simulink model "StarshipSystemModel"  (R2025b)
settings: Solver=VariableStepAuto  StartTime=0.0  StopTime=10.0  RelTol=1e-3
model workspace (MAT data in the model file):
  ActiveGNCMode : Simulink.Bus (value not decoded)
  AerodynamicControlCommand : Simulink.Bus (value not decoded)
  AerodynamicLoad : Simulink.Bus (value not decoded)
  AggregatedStream : Simulink.Bus (value not decoded)
  AllocatedEffectorDemand : Simulink.Bus (value not decoded)
  AttitudeControlDemand : Simulink.Bus (value not decoded)
  AttitudeGuidanceCommand : Simulink.Bus (value not decoded)
  AttitudeRateState : Simulink.Bus (value not decoded)
  AutogenousPressurantGas : Simulink.ConnectionBus (value not decoded)
  CandidateFaultIndication : Simulink.Bus (value not decoded)
  CombustionGasFeed : Simulink.ConnectionBus (value not decoded)
  CommandPathHealth : Simulink.Bus (value not decoded)
  ControlMode : Simulink.ValueType (value not decoded)
  DownlinkSignal : Simulink.Bus (value not decoded)
  ElectricalPower : Simulink.ConnectionBus (value not decoded)
  EngineTelemetry : Simulink.Bus (value not decoded)
  ExecutionContext : Simulink.Bus (value not decoded)
  FaultDiagnosisResult : Simulink.Bus (value not decoded)
  GNCDataContext : Simulink.Bus (value not decoded)
  GNCHealthState : Simulink.Bus (value not decoded)
  GNCStateEstimate : Simulink.Bus (value not decoded)
  GimbalAngle : Simulink.ValueType (value not decoded)
  GimbalMotion : Simulink.ConnectionBus (value not decoded)
  GroundCheckoutLink : Simulink.Bus (value not decoded)
  GroundPressurantSupply : Simulink.ConnectionBus (value not decoded)
  GuidanceConstraints : Simulink.Bus (value not decoded)
  GuidanceMode : Simulink.ValueType (value not decoded)
  LinkHealth : Simulink.Bus (value not decoded)
  LiquidPropellantFeed : Simulink.ConnectionBus (value not decoded)
  MechanicalMotion : Simulink.ConnectionBus (value not decoded)
  MechanismPosition : Simulink.Bus (value not decoded)
  ModeTransitionContext : Simulink.Bus (value not decoded)
  NavigationAidingData : Simulink.Bus (value not decoded)
  NavigationEstimate : Simulink.Bus (value not decoded)
  NavigationHealthStatus : Simulink.Bus (value not decoded)
  NavigationMeasurementSet : Simulink.Bus (value not decoded)
  PercentThrottle : Simulink.ValueType (value not decoded)
  PneumaticActuationGas : Simulink.ConnectionBus (value not decoded)
  PowerConversionStatus : Simulink.Bus (value not decoded)
  PowerDistributionStatus : Simulink.Bus (value not decoded)
  PowerHealthStatus : Simulink.Bus (value not decoded)
  PowerManagementCommand : Simulink.Bus (value not decoded)
  PowerStorageStatus : Simulink.Bus (value not decoded)
  ProtectedThermalState : Simulink.Bus (value not decoded)
  ProtectionIsolationStatus : Simulink.Bus (value not decoded)
  PurgeGasSupply : Simulink.ConnectionBus (value not decoded)
  RCSPulseCommand : Simulink.Bus (value not decoded)
  RCSTelemetry : Simulink.Bus (value not decoded)
  RFFeed : Simulink.ConnectionBus (value not decoded)
  RecoveryMechanismCommand : Simulink.Bus (value not decoded)
  RollThrottleBias : Simulink.ValueType (value not decoded)
  SafetyOverride : Simulink.ValueType (value not decoded)
  SafetyStateStatus : Simulink.Bus (value not decoded)
  ShapedControlDemand : Simulink.Bus (value not decoded)
  SpinStartIgniterGas : Simulink.ConnectionBus (value not decoded)
  StageMechanicalBoundary : Simulink.ConnectionBus (value not decoded)
  StructuralLoad : Simulink.ConnectionBus (value not decoded)
  StructureHealthStatus : Simulink.Bus (value not decoded)
  SubsystemHealthEvidence : Simulink.Bus (value not decoded)
  SubsystemStatusTelemetry : Simulink.Bus (value not decoded)
  TankTelemetry : Simulink.Bus (value not decoded)
  ThermalMonitoringCommand : Simulink.Bus (value not decoded)
  ThermalNetwork : Simulink.ConnectionBus (value not decoded)
  ThrustLoad : Simulink.ConnectionBus (value not decoded)
  TrajectoryGuidanceCommand : Simulink.Bus (value not decoded)
  TrajectoryReference : Simulink.Bus (value not decoded)
  TranslationalControlDemand : Simulink.Bus (value not decoded)
  TranslationalState : Simulink.Bus (value not decoded)
  UplinkSignal : Simulink.Bus (value not decoded)
  ValidatedControlDemand : Simulink.Bus (value not decoded)
  ValveCommand : Simulink.ValueType (value not decoded)
  VehicleStructureState : Simulink.Bus (value not decoded)
  VerifiedCommand : Simulink.Bus (value not decoded)
  VideoStream : Simulink.Bus (value not decoded)
undefined symbols (not defined in the file): ACR, ACT, ASM, ATM, BCR, BDQ, BDR, BDX, BEC, BFC, BHV, BIP, BLM, BNZ, BPI, BPR, BPV, BRX, BSM, BTA, BTP, BVC, BVE, BVV, CAA, CAM, CAS, CAT, CLM, COM, CRS, CTL, CTR, DAQ, ESC, EXT, FCR, FDB, FDE, FEX, FHI, FHM, FIC, FIS, FMG, FSC, GAP, GCM, GMD, GNC, GND, GPH, GTR, HDN, HIA, HSI, IF, INT, LOC, NAI ... (+45)
(part 8 of 8)

== system StarshipSystemModel/Starship/Propulsion/Booster main engines/Engine controller ==
  Bus Element In1 : Inport  PortName=IF-GNC-BEC-01
  Bus Element In2 : Inport  Port=2  PortName=IF-SAF-BEC-01
  IF-PWR-BEC-01 : PMIOPort  Side=Left  ConnectionType=Bus: ElectricalPower
  Bus Element Out1 : Outport  PortName=IF-BEC-SAF-01
  Bus Element Out2 : Outport  Port=2  PortName=IF-BEC-BTA-01
  Bus Element Out3 : Outport  Port=3  PortName=IF-BEC-BVC-01

== system StarshipSystemModel/Starship/Propulsion/Booster main engines/Ignition system ==
  IF-BIG-BPB-01 : PMIOPort  Side=Right
  IF-BSG-BIG-01 : PMIOPort  Port=2  Side=Left  ConnectionType=Bus: SpinStartIgniterGas

== system StarshipSystemModel/Starship/Propulsion/Booster main engines/Mounting interface ==
  IF-GMB-BMT-01 : PMIOPort  Side=Left  ConnectionType=Bus: GimbalMotion
  IF-BMT-TLI-01 : PMIOPort  Port=2  Side=Right  ConnectionType=Bus: StructuralLoad

== system StarshipSystemModel/Starship/Propulsion/Booster main engines/Nozzle ==
  IF-BCC-BNZ-01 : PMIOPort  Side=Left  ConnectionType=Bus: CombustionGasFeed
  Bus Element Out1 : Outport  PortName=IF-BNZ-BTP-01

== system StarshipSystemModel/Starship/Propulsion/Booster main engines/Preburners ==
  IF-BTP-BPB-01 : PMIOPort  Side=Left  ConnectionType=Bus: CombustionGasFeed
  IF-BPB-BCC-01 : PMIOPort  Port=2  Side=Right  ConnectionType=Bus: CombustionGasFeed
  IF-BIG-BPB-01 : PMIOPort  Port=3  Side=Left

== system StarshipSystemModel/Starship/Propulsion/Booster main engines/Turbopumps ==
  IF-BDM-BTP-01 : PMIOPort  Side=Left  ConnectionType=Bus: LiquidPropellantFeed
  IF-BVC-BTP-01 : PMIOPort  Port=2  Side=Left  ConnectionType=Bus: LiquidPropellantFeed
  IF-BTP-BPR-01 : PMIOPort  Port=3  Side=Right  ConnectionType=Bus: AutogenousPressurantGas
  IF-BTP-BPB-01 : PMIOPort  Port=4  Side=Right  ConnectionType=Bus: CombustionGasFeed

== system StarshipSystemModel/Starship/Propulsion/Booster main engines/Valves & control ==
  Bus Element In1 : Inport  PortName=IF-BEC-BVC-01
  IF-BVC-BTP-01 : PMIOPort  Side=Right  ConnectionType=Bus: LiquidPropellantFeed
  IF-BNG-BVC-01 : PMIOPort  Port=2  Side=Left  ConnectionType=Bus: PneumaticActuationGas

== system StarshipSystemModel/Starship/Propulsion/Gimbal // TVC actuation/Gimbal bearing ==
  IF-YAC-GMB-01 : PMIOPort  Side=Left  ConnectionType=Bus: GimbalMotion
  IF-PAC-GMB-01 : PMIOPort  Port=2  Side=Left  ConnectionType=Bus: GimbalMotion
  IF-GMB-BMT-01 : PMIOPort  Port=3  Side=Right  ConnectionType=Bus: GimbalMotion
  IF-GMB-SMT-01 : PMIOPort  Port=4  Side=Right  ConnectionType=Bus: GimbalMotion

== system StarshipSystemModel/Starship/Propulsion/Gimbal // TVC actuation/Pitch actuator ==
  Bus Element In1 : Inport  PortName=IF-TVC-PAC-01
  IF-PAC-GMB-01 : PMIOPort  Side=Right  ConnectionType=Bus: GimbalMotion

== system StarshipSystemModel/Starship/Propulsion/Gimbal // TVC actuation/TVC controller ==
  Bus Element In1 : Inport  PortName=IF-GNC-TVC-01
  IF-PWR-TVC-01 : PMIOPort  Side=Left  ConnectionType=Bus: ElectricalPower
  Bus Element Out1 : Outport  PortName=IF-TVC-GNC-01
  Bus Element Out3 : Outport  Port=2  PortName=IF-TVC-YAC-01
  Bus Element Out2 : Outport  Port=3  PortName=IF-TVC-PAC-01

== system StarshipSystemModel/Starship/Propulsion/Gimbal // TVC actuation/Yaw actuator ==
  Bus Element In1 : Inport  PortName=IF-TVC-YAC-01
  IF-YAC-GMB-01 : PMIOPort  Side=Right  ConnectionType=Bus: GimbalMotion

== system StarshipSystemModel/Starship/Propulsion/RCS thrusters/Igniter ==
  IF-RIG-RTC-01 : PMIOPort  Side=Right

== system StarshipSystemModel/Starship/Propulsion/RCS thrusters/RCS controller ==
  Bus Element In1 : Inport  PortName=IF-GNC-RCT-01
  IF-PWR-RCT-01 : PMIOPort  Side=Left  ConnectionType=Bus: ElectricalPower
  Bus Element Out1 : Outport  PortName=IF-RCT-SAF-01
  Bus Element Out2 : Outport  Port=2  PortName=IF-RCT-RVM-01

== system StarshipSystemModel/Starship/Propulsion/RCS thrusters/Thruster chamber, nozzle ==
  IF-RVM-RTC-01 : PMIOPort  Side=Left  ConnectionType=Bus: CombustionGasFeed
  IF-RIG-RTC-01 : PMIOPort  Port=2  Side=Left

== system StarshipSystemModel/Starship/Propulsion/RCS thrusters/Valve & feed manifold ==
  Bus Element In1 : Inport  PortName=IF-RCT-RVM-01
  IF-SPR-RVM-01 : PMIOPort  Side=Left  ConnectionType=Bus: CombustionGasFeed
  IF-RVM-RTC-01 : PMIOPort  Port=2  Side=Right  ConnectionType=Bus: CombustionGasFeed

== system StarshipSystemModel/Starship/Propulsion/Ship main engines/Combustion Chamber  ==
  IF-SPB-SCC-01 : PMIOPort  Side=Left  ConnectionType=Bus: CombustionGasFeed
  IF-SCC-SNZ-01 : PMIOPort  Port=2  Side=Right  ConnectionType=Bus: CombustionGasFeed

== system StarshipSystemModel/Starship/Propulsion/Ship main engines/Engine controller ==
  Bus Element In1 : Inport  PortName=IF-GNC-SEC-01
  Bus Element In2 : Inport  Port=2  PortName=IF-SAF-SEC-01
  IF-PWR-SEC-01 : PMIOPort  Side=Left  ConnectionType=Bus: ElectricalPower
  Bus Element Out1 : Outport  PortName=IF-SEC-SAF-01
  Bus Element Out2 : Outport  Port=2  PortName=IF-SEC-STA-01
  Bus Element Out3 : Outport  Port=3  PortName=IF-SEC-SVC-01

== system StarshipSystemModel/Starship/Propulsion/Ship main engines/Ignition system ==
  IF-SIG-SPB-01 : PMIOPort  Side=Right
  IF-SSG-SIG-01 : PMIOPort  Port=2  Side=Left  ConnectionType=Bus: SpinStartIgniterGas

== system StarshipSystemModel/Starship/Propulsion/Ship main engines/Mounting interface ==
  IF-GMB-SMT-01 : PMIOPort  Side=Left  ConnectionType=Bus: GimbalMotion
  IF-SMT-TLI-01 : PMIOPort  Port=2  Side=Right  ConnectionType=Bus: StructuralLoad

== system StarshipSystemModel/Starship/Propulsion/Ship main engines/Nozzle ==
  IF-SCC-SNZ-01 : PMIOPort  Side=Left  ConnectionType=Bus: CombustionGasFeed
  Bus Element Out1 : Outport  PortName=IF-SNZ-STP-01

== system StarshipSystemModel/Starship/Propulsion/Ship main engines/Preburners ==
  IF-STP-SPB-01 : PMIOPort  Side=Left  ConnectionType=Bus: CombustionGasFeed
  IF-SIG-SPB-01 : PMIOPort  Port=2  Side=Left
  IF-SPB-SCC-01 : PMIOPort  Port=3  Side=Right  ConnectionType=Bus: CombustionGasFeed

== system StarshipSystemModel/Starship/Propulsion/Ship main engines/Turbopumps ==
  IF-SDM-STP-01 : PMIOPort  Side=Left  ConnectionType=Bus: LiquidPropellantFeed
  IF-SVC-STP-01 : PMIOPort  Port=2  Side=Left  ConnectionType=Bus: LiquidPropellantFeed
  IF-STP-SPR-01 : PMIOPort  Port=3  Side=Right  ConnectionType=Bus: AutogenousPressurantGas
  IF-STP-SPB-01 : PMIOPort  Port=4  Side=Right  ConnectionType=Bus: CombustionGasFeed

== system StarshipSystemModel/Starship/Propulsion/Ship main engines/Valves & control ==
  Bus Element In1 : Inport  PortName=IF-SEC-SVC-01
  IF-SVC-STP-01 : PMIOPort  Side=Right  ConnectionType=Bus: LiquidPropellantFeed
  IF-SNG-SVC-01 : PMIOPort  Port=2  Side=Left  ConnectionType=Bus: PneumaticActuationGas

== system StarshipSystemModel/Starship/Safety & Fault Management /Fault Diagnosis & Isolation/Fault Correlation & Reasoning ==
  Bus Element In1 : Inport  PortName=IF-FDE-FCR-01
  Bus Element Out1 : Outport  PortName=IF-FCR-FIS-01

== system StarshipSystemModel/Starship/Safety & Fault Management /Fault Diagnosis & Isolation/Fault Identification & Classification ==
  Bus Element In1 : Inport  PortName=IF-FIS-FIC-01
  Bus Element Out1 : Outport  PortName=IF-FIC-SEA-01

== system StarshipSystemModel/Starship/Safety & Fault Management /Fault Diagnosis & Isolation/Fault Isolation ==
  Bus Element In1 : Inport  PortName=IF-FCR-FIS-01
  Bus Element Out1 : Outport  PortName=IF-FIS-FIC-01

== system StarshipSystemModel/Starship/Safety & Fault Management /Fault Management & Response Logic/Protective Action Coordination ==
  Bus Element In1 : Inport  PortName=IF-RSL-PAC-01
  Bus Element Out1 : Outport  PortName=IF-SAF-BEC-01
  Bus Element Out2 : Outport  Port=2  PortName=IF-SAF-SEC-01
  Bus Element Out3 : Outport  Port=3  PortName=IF-PAC-RCO-01

== system StarshipSystemModel/Starship/Safety & Fault Management /Fault Management & Response Logic/Response Selection Logic ==
  Bus Element In1 : Inport  PortName=IF-SEA-RSL-01
  Bus Element Out1 : Outport  PortName=IF-RSL-PAC-01

== system StarshipSystemModel/Starship/Safety & Fault Management /Fault Management & Response Logic/Severity & Consequence Assessment ==
  Bus Element In1 : Inport  PortName=IF-FIC-SEA-01
  Bus Element Out1 : Outport  PortName=IF-SEA-RSL-01

== system StarshipSystemModel/Starship/Safety & Fault Management /Health Monitoring & Fault Detection/Fault Detection Engine ==
  Bus Element In1 : Inport  PortName=IF-VIE-FDE-01
  Bus Element Out1 : Outport  PortName=IF-FDE-FCR-01

== system StarshipSystemModel/Starship/Safety & Fault Management /Health Monitoring & Fault Detection/Health Information Aggregation ==
  Bus Element In11 : Inport  PortName=IF-RSM-SAF-01
  Bus Element In10 : Inport  Port=2  PortName=IF-INT-SAF-01
  Bus Element In9 : Inport  Port=3  PortName=IF-POS-SAF-01
  Bus Element In8 : Inport  Port=4  PortName=IF-TMS-SAF-01
  Bus Element In7 : Inport  Port=5  PortName=IF-FHM-SAF-01
  Bus Element In1 : Inport  Port=6  PortName=IF-BEC-SAF-01
  Bus Element In2 : Inport  Port=7  PortName=IF-SEC-SAF-01
  Bus Element In3 : Inport  Port=8  PortName=IF-RCT-SAF-01
  Bus Element In4 : Inport  Port=9  PortName=IF-BPR-SAF-01
  Bus Element In5 : Inport  Port=10  PortName=IF-SPR-SAF-01
  Bus Element In6 : Inport  Port=11  PortName=IF-PMM-SAF-01
  Bus Element In12 : Inport  Port=12  PortName=IF-BLM-SAF-01
  Bus Element In13 : Inport  Port=13  PortName=IF-SLM-SAF-01
  Bus Element In14 : Inport  Port=14  PortName=IF-ESC-HIA-01
  Bus Element Out1 : Outport  PortName=IF-HIA-VIE-01

== system StarshipSystemModel/Starship/Safety & Fault Management /Health Monitoring & Fault Detection/Validity & Integrity Evaluation ==
  Bus Element In1 : Inport  PortName=IF-HIA-VIE-01
  Bus Element Out1 : Outport  PortName=IF-VIE-FDE-01

== system StarshipSystemModel/Starship/Safety & Fault Management /Recovery & Reconfiguration Management/Reconfiguration Coordinator ==
  Bus Element In1 : Inport  PortName=IF-PAC-RCO-01
  Bus Element Out1 : Outport  PortName=IF-RCO-RSE-01

== system StarshipSystemModel/Starship/Safety & Fault Management /Recovery & Reconfiguration Management/Recovery Sequence Executor ==
  Bus Element In1 : Inport  PortName=IF-RCO-RSE-01
  Bus Element Out1 : Outport  PortName=IF-SAF-RSM-01
  Bus Element Out2 : Outport  Port=2  PortName=IF-RSE-RVF-01

== system StarshipSystemModel/Starship/Safety & Fault Management /Recovery & Reconfiguration Management/Recovery Verification ==
  Bus Element In1 : Inport  PortName=IF-RSE-RVF-01
  Bus Element Out1 : Outport  PortName=IF-RVF-SSM-01

== system StarshipSystemModel/Starship/Safety & Fault Management /Safety State & Flight-Safety Management/Escalation & Containment Status ==
  Bus Element In1 : Inport  PortName=IF-FSC-ESC-01
  Bus Element Out2 : Outport  PortName=IF-SAF-STA-01
  Bus Element Out1 : Outport  Port=2  PortName=IF-SAF-BTA-01
  Bus Element Out3 : Outport  Port=3  PortName=IF-ESC-HIA-01

== system StarshipSystemModel/Starship/Safety & Fault Management /Safety State & Flight-Safety Management/Flight-Safety Coordination ==
  Bus Element In1 : Inport  PortName=IF-BCR-SAF-01
  Bus Element In2 : Inport  Port=2  PortName=IF-SCR-SAF-01
  Bus Element In3 : Inport  Port=3  PortName=IF-SSM-FSC-01
  Bus Element Out1 : Outport  PortName=IF-FSC-ESC-01

== system StarshipSystemModel/Starship/Safety & Fault Management /Safety State & Flight-Safety Management/Safety State Manager ==
  Bus Element In1 : Inport  PortName=IF-RVF-SSM-01
  Bus Element Out1 : Outport  PortName=IF-SAF-FHM-01
  Bus Element Out2 : Outport  Port=2  PortName=IF-SSM-FSC-01

== system StarshipSystemModel/Starship/Structure and Mechanisms/Aerodynamic Control Mechanisms/Actuator ==
  Bus Element In1 : Inport  PortName=IF-GNC-ACT-01
  Bus Element In2 : Inport  Port=2  PortName=IF-POS-ACT-01
  IF-ACT-HNG-01 : PMIOPort  Side=Right  ConnectionType=Bus: MechanicalMotion
  IF-PWR-STR-01 : PMIOPort  Port=2  Side=Left  ConnectionType=Bus: ElectricalPower

== system StarshipSystemModel/Starship/Structure and Mechanisms/Aerodynamic Control Mechanisms/Hinge // linkage ==
  IF-SUR-HNG-01 : PMIOPort  Side=Left  ConnectionType=Bus: MechanicalMotion
  IF-ACT-HNG-01 : PMIOPort  Port=2  Side=Left  ConnectionType=Bus: MechanicalMotion
  IF-HNG-SUR-01 : PMIOPort  Port=3  Side=Right
  IF-HNG-INT-01 : PMIOPort  Port=4  Side=Right

== system StarshipSystemModel/Starship/Structure and Mechanisms/Aerodynamic Control Mechanisms/Position // health ==
  Bus Element Out1 : Outport  PortName=IF-POS-GNC-01
  Bus Element Out2 : Outport  Port=2  PortName=IF-POS-ACT-01
  Bus Element Out3 : Outport  Port=3  PortName=IF-POS-SAF-01

== system StarshipSystemModel/Starship/Structure and Mechanisms/Aerodynamic Control Mechanisms/Surface // fin // flap ==
  Bus Element In1 : Inport  PortName=IF-ATM-SUR-01
  IF-HNG-SUR-01 : PMIOPort  Side=Left
  IF-SUR-HNG-01 : PMIOPort  Port=2  Side=Right  ConnectionType=Bus: MechanicalMotion

== system StarshipSystemModel/Starship/Structure and Mechanisms/Primary Load-Bearing Airframe/ Load-transfer structure ==
  IF-PRS-LDT-01 : PMIOPort  Side=Left
  IF-LDT-INT-01 : PMIOPort  Port=2  Side=Right
  IF-TLI-LDT-01 : PMIOPort  Port=3  Side=Left

== system StarshipSystemModel/Starship/Structure and Mechanisms/Primary Load-Bearing Airframe/Local interface structure ==
  IF-LDT-INT-01 : PMIOPort  Side=Left
  IF-INT-PRS-01 : PMIOPort  Port=2  Side=Right
  IF-SLS-LDT-01 : PMIOPort  Port=3  Side=Left
  IF-HNG-INT-01 : PMIOPort  Port=4  Side=Left
  Bus Element Out3 : Outport  PortName=IF-INT-SAF-01
  Bus Element Out1 : Outport  Port=2  PortName=IF-INT-STA-01
  Bus Element Out2 : Outport  Port=3  PortName=IF-INT-BTA-01

== system StarshipSystemModel/Starship/Structure and Mechanisms/Primary Load-Bearing Airframe/Primary pressure//shell ==
  IF-BOT-PRS-01 : PMIOPort  Side=Right  ConnectionType=Bus: StructuralLoad
  IF-SOT-PRS-01 : PMIOPort  Port=2  Side=Right  ConnectionType=Bus: StructuralLoad
  IF-RLI-PRS-01 : PMIOPort  Port=3  Side=Left
  IF-TBI-PRS-01 : PMIOPort  Port=4  Side=Left  ConnectionType=Bus: ThermalNetwork
  IF-BTP-PRS-01 : PMIOPort  Port=5  Side=Left  ConnectionType=Bus: ThermalNetwork
  IF-STP-PRS-01 : PMIOPort  Port=6  Side=Left  ConnectionType=Bus: ThermalNetwork
  IF-PRS-LDT-01 : PMIOPort  Port=7  Side=Right
  IF-INT-PRS-01 : PMIOPort  Port=8  Side=Left

== system StarshipSystemModel/Starship/Structure and Mechanisms/Recovery & Landing Mechanisms/Landing//catch load path ==
  IF-RLI-GND-01 : PMIOPort  Side=Right  ConnectionType=Bus: StructuralLoad
  IF-RME-RLI-01 : PMIOPort  Port=2  Side=Left  ConnectionType=Bus: MechanicalMotion
  IF-RLI-PRS-01 : PMIOPort  Port=3  Side=Right

== system StarshipSystemModel/Starship/Structure and Mechanisms/Recovery & Landing Mechanisms/Recovery mechanism ==
  IF-RME-RLI-01 : PMIOPort  Side=Right  ConnectionType=Bus: MechanicalMotion
  Bus Element Out1 : Outport  PortName=IF-RME-RSM-01

== system StarshipSystemModel/Starship/Structure and Mechanisms/Recovery & Landing Mechanisms/Recovery state//health ==
  Bus Element In1 : Inport  PortName=IF-RME-RSM-01
  Bus Element In2 : Inport  Port=2  PortName=IF-SAF-RSM-01
  Bus Element Out1 : Outport  PortName=IF-RSM-SAF-01

== system StarshipSystemModel/Starship/Structure and Mechanisms/Stage & Thrust Interfaces/Hot-stage interface ==
  IF-HSI-SLS-01 : PMIOPort  Side=Right  ConnectionType=Bus: StageMechanicalBoundary

== system StarshipSystemModel/Starship/Structure and Mechanisms/Stage & Thrust Interfaces/Separation response ==
  IF-HSI-SLS-01 : PMIOPort  Side=Left  ConnectionType=Bus: StageMechanicalBoundary
  IF-SLS-LDT-01 : PMIOPort  Port=2  Side=Right

== system StarshipSystemModel/Starship/Structure and Mechanisms/Stage & Thrust Interfaces/Thrust-load introduction ==
  IF-BMT-TLI-01 : PMIOPort  Side=Right
  IF-SMT-TLI-01 : PMIOPort  Port=2  Side=Right
  IF-TLI-LDT-01 : PMIOPort  Port=3  Side=Right

== system StarshipSystemModel/Starship/Thermal Protection/Ship Primary TPS/Base heat-shield region ==

== system StarshipSystemModel/Starship/Thermal Protection/Ship Primary TPS/Control-surface thermal protection ==
  Bus Element Out1 : Outport  PortName=IF-STP-CTL-TBI-CTL-01

== system StarshipSystemModel/Starship/Thermal Protection/Ship Primary TPS/Localized high-heating protection ==
  Bus Element Out1 : Outport  PortName=IF-STP-LOC-TBI-STP-01

== system StarshipSystemModel/Starship/Thermal Protection/Ship Primary TPS/Primary TPS acreage // tile field ==
  Bus Element In1 : Inport  PortName=IF-ATM-STP-01
  Bus Element In2 : Inport  Port=2  PortName=IF-SNZ-STP-01
  IF-STP-PRS-01 : PMIOPort  Side=Right  ConnectionType=Bus: ThermalNetwork
  Bus Element Out1 : Outport  PortName=IF-STP-ACR-TBI-GAP-01

== system StarshipSystemModel/Starship/Thermal Protection/Super Heavy Thermal Protection/Base heat-shield region ==

== system StarshipSystemModel/Starship/Thermal Protection/Super Heavy Thermal Protection/Forward heat-shield // interstage ==
  Bus Element Out1 : Outport  PortName=IF-BTP-FHI-TBI-INT-01

== system StarshipSystemModel/Starship/Thermal Protection/Super Heavy Thermal Protection/Localized thermal protection ==
  IF-BTP-PRS-01 : PMIOPort  Side=Right  ConnectionType=Bus: ThermalNetwork
  Bus Element Out1 : Outport  PortName=IF-BTP-LOC-TBI-STP-01

== system StarshipSystemModel/Starship/Thermal Protection/Super Heavy Thermal Protection/Primary TPS acreage ==
  Bus Element In1 : Inport  PortName=IF-BNZ-BTP-01
  Bus Element In2 : Inport  Port=2  PortName=IF-ATM-BTP-01
  Bus Element Out1 : Outport  PortName=IF-BTP-ACR-TBI-GAP-01

== system StarshipSystemModel/Starship/Thermal Protection/Thermal Barriers & Discontinuity Protection/Control-surface boundary // closeout protection ==
  Bus Element In1 : Inport  PortName=IF-STP-CTL-TBI-CTL-01
  Bus Element Out1 : Outport  PortName=IF-TBI-CTL-TMS-SNS-01

== system StarshipSystemModel/Starship/Thermal Protection/Thermal Barriers & Discontinuity Protection/Penetration and interface barriers ==
  Bus Element In1 : Inport  PortName=IF-BTP-FHI-TBI-INT-01
  Bus Element Out1 : Outport  PortName=IF-TBI-INT-TMS-SNS-01

== system StarshipSystemModel/Starship/Thermal Protection/Thermal Barriers & Discontinuity Protection/Step // protrusion thermal management ==
  Bus Element In2 : Inport  PortName=IF-BTP-LOC-TBI-STP-01
  Bus Element In1 : Inport  Port=2  PortName=IF-STP-LOC-TBI-STP-01
  IF-TBI-PRS-01 : PMIOPort  Side=Right  ConnectionType=Bus: ThermalNetwork

== system StarshipSystemModel/Starship/Thermal Protection/Thermal Barriers & Discontinuity Protection/Tile-gap // seam thermal protection ==
  Bus Element In2 : Inport  PortName=IF-BTP-ACR-TBI-GAP-01
  Bus Element In1 : Inport  Port=2  PortName=IF-STP-ACR-TBI-GAP-01
  Bus Element Out1 : Outport  PortName=IF-TBI-GAP-TMS-SNS-01

== system StarshipSystemModel/Starship/Thermal Protection/Thermal Monitoring & Assessment/External thermal-observation data interface ==
  Bus Element Out1 : Outport  PortName=IF-TMS-EXT-ASM-01

== system StarshipSystemModel/Starship/Thermal Protection/Thermal Monitoring & Assessment/TPS thermal sensors ==
  Bus Element In1 : Inport  PortName=IF-TBI-GAP-TMS-SNS-01
  Bus Element In2 : Inport  Port=2  PortName=IF-TBI-INT-TMS-SNS-01
  Bus Element In3 : Inport  Port=3  PortName=IF-TBI-CTL-TMS-SNS-01
  Bus Element In4 : Inport  Port=4  PortName=IF-GNC-TMS-01
  IF-PWR-TMS-01 : PMIOPort  Side=Left  ConnectionType=Bus: ElectricalPower
  Bus Element Out1 : Outport  PortName=IF-TMS-SNS-DAQ-01

== system StarshipSystemModel/Starship/Thermal Protection/Thermal Monitoring & Assessment/Thermal assessment // reconstruction function ==
  Bus Element In1 : Inport  PortName=IF-TMS-DAQ-ASM-01
  Bus Element In2 : Inport  Port=2  PortName=IF-TMS-EXT-ASM-01
  Bus Element Out1 : Outport  PortName=IF-TMS-ASM-DAQ-01

== system StarshipSystemModel/Starship/Thermal Protection/Thermal Monitoring & Assessment/Thermal-data acquisition // telemetry path ==
  Bus Element In1 : Inport  PortName=IF-TMS-SNS-DAQ-01
  Bus Element In3 : Inport  Port=2  PortName=IF-TMS-ASM-DAQ-01
  Bus Element Out1 : Outport  PortName=IF-TMS-DAQ-ASM-01

== system StarshipSystemModel/Starship/Communications/Booster/Command & Data Handling (C&DH)/Command decoder & router ==
  Bus Element In2 : Inport  PortName=IF-BDQ-BCR-01
  Bus Element In1 : Inport  Port=2  PortName=IF-BLM-BCR-01
  Bus Element Out1 : Outport  PortName=IF-BCR-GNC-01
  Bus Element Out2 : Outport  Port=2  PortName=IF-BCR-SAF-01

== system StarshipSystemModel/Starship/Communications/Booster/Command & Data Handling (C&DH)/Data recorder (mass memory) ==
  Bus Element In1 : Inport  PortName=IF-BTA-BDR-01

== system StarshipSystemModel/Starship/Communications/Booster/Command & Data Handling (C&DH)/Link management controller ==
  Bus Element In1 : Inport  PortName=IF-BTA-BLM-01
  Bus Element In2 : Inport  Port=2  PortName=IF-BRX-BLM-01
  Bus Element In3 : Inport  Port=3  PortName=IF-BDX-BLM-01
  Bus Element Out1 : Outport  PortName=IF-BLM-SAF-01
  Bus Element Out2 : Outport  Port=2  PortName=IF-BLM-BRX-01
  Bus Element Out3 : Outport  Port=3  PortName=IF-BLM-BDX-01
  Bus Element Out4 : Outport  Port=4  PortName=IF-BLM-BCR-01

== system StarshipSystemModel/Starship/Communications/Booster/Command & Data Handling (C&DH)/Telemetry aggregator ==
  Bus Element In6 : Inport  PortName=IF-INT-BTA-01
  Bus Element In5 : Inport  Port=2  PortName=IF-TMS-BTA-01
  Bus Element In3 : Inport  Port=3  PortName=IF-GNC-BTA-01
  Bus Element In1 : Inport  Port=4  PortName=IF-BEC-BTA-01
  Bus Element In2 : Inport  Port=5  PortName=IF-BPR-BTA-01
  Bus Element In7 : Inport  Port=6  PortName=IF-BVE-BTA-01
  Bus Element In4 : Inport  Port=7  PortName=IF-SAF-BTA-01
  IF-PWR-BTA-01 : PMIOPort  Side=Left  ConnectionType=Bus: ElectricalPower
  Bus Element Out1 : Outport  PortName=IF-BTA-BLM-01
  Bus Element Out2 : Outport  Port=2  PortName=IF-BTA-BDR-01
  Bus Element Out3 : Outport  Port=3  PortName=IF-BTA-BDQ-01

== system StarshipSystemModel/Starship/Communications/Booster/Command & Data Handling (C&DH)/Video capture & encoding ==
  Bus Element Out1 : Outport  PortName=IF-BVE-BTA-01

== system StarshipSystemModel/Starship/Communications/Booster/Direct-to-ground RF terminal/Antenna array ==
  IF-BDA-BDX-01 : PMIOPort  Side=Right  ConnectionType=Bus: RFFeed

== system StarshipSystemModel/Starship/Communications/Booster/Direct-to-ground RF terminal/RF transceiver unit ==
  Bus Element In1 : Inport  PortName=IF-GND-BDX-01
  Bus Element In2 : Inport  Port=2  PortName=IF-BLM-BDX-01
  IF-PWR-BDX-01 : PMIOPort  Side=Left  ConnectionType=Bus: ElectricalPower
  IF-BDA-BDX-01 : PMIOPort  Port=2  Side=Left  ConnectionType=Bus: RFFeed
  Bus Element Out1 : Outport  PortName=IF-BDX-GND-01
  Bus Element Out2 : Outport  Port=2  PortName=IF-BDX-BLM-01

== system StarshipSystemModel/Starship/Communications/Booster/Ground data interface/Vehicle-side data QD panel ==
  Bus Element In2 : Inport  PortName=IF-BTA-BDQ-01
  Bus Element In1 : Inport  Port=2  PortName=IF-GND-BDQ-01
  Bus Element Out1 : Outport  PortName=IF-BDQ-GND-01
  Bus Element Out2 : Outport  Port=2  PortName=IF-BDQ-BCR-01

== system StarshipSystemModel/Starship/Communications/Booster/Relay link terminal/Antenna aperture & radome ==
  IF-BRA-BRX-01 : PMIOPort  Side=Right  ConnectionType=Bus: RFFeed
  IF-PWR-BRA-01 : PMIOPort  Port=2  Side=Left  ConnectionType=Bus: ElectricalPower

== system StarshipSystemModel/Starship/Communications/Booster/Relay link terminal/RF//optical transceiver unit ==
  Bus Element In1 : Inport  PortName=IF-GND-BRX-01
  Bus Element In2 : Inport  Port=2  PortName=IF-BLM-BRX-01
  IF-BRA-BRX-01 : PMIOPort  Side=Left  ConnectionType=Bus: RFFeed
  IF-PWR-BRX-01 : PMIOPort  Port=2  Side=Left  ConnectionType=Bus: ElectricalPower
  Bus Element Out1 : Outport  PortName=IF-BRX-GND-01
  Bus Element Out2 : Outport  Port=2  PortName=IF-BRX-BLM-01

== system StarshipSystemModel/Starship/Communications/Ship/Command & Data Handling (C&DH)/Command decoder & router ==
  Bus Element In2 : Inport  PortName=IF-SDQ-SCR-01
  Bus Element In1 : Inport  Port=2  PortName=IF-SLM-SCR-01
  Bus Element Out1 : Outport  PortName=IF-SCR-GNC-01
  Bus Element Out2 : Outport  Port=2  PortName=IF-SCR-SAF-01

== system StarshipSystemModel/Starship/Communications/Ship/Command & Data Handling (C&DH)/Data recorder (mass memory) ==
  Bus Element In1 : Inport  PortName=IF-STA-SDR-01

== system StarshipSystemModel/Starship/Communications/Ship/Command & Data Handling (C&DH)/Link management controller ==
  Bus Element In1 : Inport  PortName=IF-STA-SLM-01
  Bus Element In2 : Inport  Port=2  PortName=IF-SRX-SLM-01
  Bus Element In3 : Inport  Port=3  PortName=IF-SDX-SLM-01
  Bus Element Out1 : Outport  PortName=IF-SLM-SAF-01
  Bus Element Out2 : Outport  Port=2  PortName=IF-SLM-SRX-01
  Bus Element Out3 : Outport  Port=3  PortName=IF-SLM-SDX-01
  Bus Element Out4 : Outport  Port=4  PortName=IF-SLM-SCR-01

== system StarshipSystemModel/Starship/Communications/Ship/Command & Data Handling (C&DH)/Telemetry aggregator ==
  Bus Element In5 : Inport  PortName=IF-TMS-STA-01
  Bus Element In3 : Inport  Port=2  PortName=IF-GNC-STA-01
  Bus Element In1 : Inport  Port=3  PortName=IF-SEC-STA-01
  Bus Element In2 : Inport  Port=4  PortName=IF-SPR-STA-01
  Bus Element In7 : Inport  Port=5  PortName=IF-SVE-STA-01
  Bus Element In4 : Inport  Port=6  PortName=IF-SAF-STA-01
  Bus Element In6 : Inport  Port=7  PortName=IF-INT-STA-01
  IF-PWR-STA-01 : PMIOPort  Side=Left  ConnectionType=Bus: ElectricalPower
  Bus Element Out1 : Outport  PortName=IF-STA-SLM-01
  Bus Element Out2 : Outport  Port=2  PortName=IF-STA-SDR-01
  Bus Element Out3 : Outport  Port=3  PortName=IF-STA-SDQ-01

== system StarshipSystemModel/Starship/Communications/Ship/Command & Data Handling (C&DH)/Video capture & encoding ==
  Bus Element Out1 : Outport  PortName=IF-SVE-STA-01

== system StarshipSystemModel/Starship/Communications/Ship/Direct-to-ground RF terminal/Antenna array ==
  IF-SDA-SDX-01 : PMIOPort  Side=Right  ConnectionType=Bus: RFFeed

== system StarshipSystemModel/Starship/Communications/Ship/Direct-to-ground RF terminal/RF transceiver unit ==
  Bus Element In1 : Inport  PortName=IF-GND-SDX-01
  Bus Element In2 : Inport  Port=2  PortName=IF-SLM-SDX-01
  IF-PWR-SDX-01 : PMIOPort  Side=Left  ConnectionType=Bus: ElectricalPower
  IF-SDA-SDX-01 : PMIOPort  Port=2  Side=Left  ConnectionType=Bus: RFFeed
  Bus Element Out1 : Outport  PortName=IF-SDX-GND-01
  Bus Element Out2 : Outport  Port=2  PortName=IF-SDX-SLM-01

== system StarshipSystemModel/Starship/Communications/Ship/Ground data interface/Vehicle-side data QD panel ==
  Bus Element In2 : Inport  PortName=IF-STA-SDQ-01
  Bus Element In1 : Inport  Port=2  PortName=IF-GND-SDQ-01
  Bus Element Out1 : Outport  PortName=IF-SDQ-GND-01
  Bus Element Out2 : Outport  Port=2  PortName=IF-SDQ-SCR-01

== system StarshipSystemModel/Starship/Communications/Ship/Relay link terminal/Antenna aperture & radome ==
  IF-SRA-SRX-01 : PMIOPort  Side=Right  ConnectionType=Bus: RFFeed
  IF-PWR-SRA-01 : PMIOPort  Port=2  Side=Left  ConnectionType=Bus: ElectricalPower
  Bus Element Out1 : Outport  PortName=IF-SRX-SLM-01

== system StarshipSystemModel/Starship/Communications/Ship/Relay link terminal/RF//optical transceiver unit ==
  Bus Element In1 : Inport  PortName=IF-GND-SRX-01
  Bus Element In2 : Inport  Port=2  PortName=IF-SLM-SRX-01
  IF-SRA-SRX-01 : PMIOPort  Side=Left  ConnectionType=Bus: RFFeed
  IF-PWR-SRX-01 : PMIOPort  Port=2  Side=Left  ConnectionType=Bus: ElectricalPower
  Bus Element Out1 : Outport  PortName=IF-SRX-GND-01

== system StarshipSystemModel/Starship/Propellent system/Booster propellant System/Booster propellant tanks/Anti-slosh baffles ==

== system StarshipSystemModel/Starship/Propellent system/Booster propellant System/Booster propellant tanks/CH4 main tank ==
  IF-BFT-BPV-01 : PMIOPort  Side=Right  ConnectionType=Bus: LiquidPropellantFeed
  IF-BCQ-BFT-01 : PMIOPort  Port=2  Side=Left  ConnectionType=Bus: LiquidPropellantFeed
  IF-BPR-BFT-01 : PMIOPort  Port=3  Side=Left  ConnectionType=Bus: AutogenousPressurantGas
  IF-BFT-BVV-01 : PMIOPort  Port=4  Side=Right  ConnectionType=Bus: AutogenousPressurantGas

== system StarshipSystemModel/Starship/Propellent system/Booster propellant System/Booster propellant tanks/CH4 transfer tube (downcomer) ==

== system StarshipSystemModel/Starship/Propellent system/Booster propellant System/Booster propellant tanks/Common dome ==

== system StarshipSystemModel/Starship/Propellent system/Booster propellant System/Booster propellant tanks/LOX landing tank ==
  IF-BLT-BHV-01 : PMIOPort  Side=Right  ConnectionType=Bus: LiquidPropellantFeed

== system StarshipSystemModel/Starship/Propellent system/Booster propellant System/Booster propellant tanks/LOX main tank ==
  IF-BOT-BPV-01 : PMIOPort  Side=Right
  IF-BOT-PRS-01 : PMIOPort  Port=2  Side=Left  ConnectionType=Bus: StructuralLoad
  IF-BPR-BOT-01 : PMIOPort  Port=3  Side=Left  ConnectionType=Bus: AutogenousPressurantGas
  IF-BOT-BVV-01 : PMIOPort  Port=4  Side=Right  ConnectionType=Bus: AutogenousPressurantGas
  IF-BLQ-BOT-01 : PMIOPort  Port=5  Side=Left  ConnectionType=Bus: LiquidPropellantFeed

== system StarshipSystemModel/Starship/Propellent system/Booster propellant System/Feed & distribution/Distribution manifold ==
  IF-BDM-BTP-01 : PMIOPort  Side=Right  ConnectionType=Bus: LiquidPropellantFeed
  IF-BHV-BDM-01 : PMIOPort  Port=2  Side=Left  ConnectionType=Bus: LiquidPropellantFeed
  IF-BPV-BDM-01 : PMIOPort  Port=3  Side=Left  ConnectionType=Bus: LiquidPropellantFeed

== system StarshipSystemModel/Starship/Propellent system/Booster propellant System/Feed & distribution/Feed controller ==
  Bus Element In1 : Inport  PortName=IF-GNC-BFC-01
  IF-PWR-BFC-01 : PMIOPort  Side=Left  ConnectionType=Bus: ElectricalPower
  Bus Element Out1 : Outport  PortName=IF-BFC-BPV-01
  Bus Element Out2 : Outport  Port=2  PortName=IF-BFC-BHV-01

== system StarshipSystemModel/Starship/Propellent system/Booster propellant System/Feed & distribution/Header tank switchover valve ==
  Bus Element In1 : Inport  PortName=IF-BFC-BHV-01
  IF-BLT-BHV-01 : PMIOPort  Side=Left  ConnectionType=Bus: LiquidPropellantFeed
  IF-BHV-BDM-01 : PMIOPort  Port=2  Side=Right  ConnectionType=Bus: LiquidPropellantFeed
  IF-BNG-BHV-01 : PMIOPort  Port=3  Side=Left  ConnectionType=Bus: PneumaticActuationGas

== system StarshipSystemModel/Starship/Propellent system/Booster propellant System/Feed & distribution/Main tank outlet valve (prevalve) ==
  Bus Element In1 : Inport  PortName=IF-BFC-BPV-01
  IF-BOT-BPV-01 : PMIOPort  Side=Left  ConnectionType=Bus: LiquidPropellantFeed
  IF-BFT-BPV-01 : PMIOPort  Port=2  Side=Left  ConnectionType=Bus: LiquidPropellantFeed
  IF-BPV-BDM-01 : PMIOPort  Port=3  Side=Right  ConnectionType=Bus: LiquidPropellantFeed
  IF-BNG-BPV-01 : PMIOPort  Port=4  Side=Left  ConnectionType=Bus: PneumaticActuationGas

== system StarshipSystemModel/Starship/Propellent system/Booster propellant System/Ground propellant interface/CH4 quick-disconnect panel ==
  "IF-GND-BCQ-01\t" : PMIOPort  Side=Left
  IF-BCQ-BFT-01 : PMIOPort  Port=2  Side=Right  ConnectionType=Bus: LiquidPropellantFeed

== system StarshipSystemModel/Starship/Propellent system/Booster propellant System/Ground propellant interface/LOX quick-disconnect panel ==
  "IF-GND-BLQ-01\t" : PMIOPort  Side=Left
  IF-BLQ-BOT-01 : PMIOPort  Port=2  Side=Right  ConnectionType=Bus: LiquidPropellantFeed

== system StarshipSystemModel/Starship/Propellent system/Booster propellant System/Ground propellant interface/Purge//pressurant ground QD ==
  IF-GND-BPQ-01 : PMIOPort  Side=Left  ConnectionType=Bus: GroundPressurantSupply
  IF-BPQ-BSG-01 : PMIOPort  Port=2  Side=Right  ConnectionType=Bus: GroundPressurantSupply
  IF-BPQ-BPR-01 : PMIOPort  Port=3  Side=Right  ConnectionType=Bus: GroundPressurantSupply
  IF-BPQ-BNG-01 : PMIOPort  Port=4  Side=Right  ConnectionType=Bus: GroundPressurantSupply

== system StarshipSystemModel/Starship/Propellent system/Booster propellant System/Pressurization, purge & venting/Autogenous pressurization regulator ==
  Bus Element In1 : Inport  PortName=IF-GNC-BPR-01
  IF-BPQ-BPR-01 : PMIOPort  Side=Left  ConnectionType=Bus: GroundPressurantSupply
  IF-BTP-BPR-01 : PMIOPort  Port=2  Side=Left  ConnectionType=Bus: AutogenousPressurantGas
  IF-BPR-BOT-01 : PMIOPort  Port=3  Side=Right  ConnectionType=Bus: AutogenousPressurantGas
  IF-BPR-BFT-01 : PMIOPort  Port=4  Side=Right  ConnectionType=Bus: AutogenousPressurantGas
  IF-PWR-BPR-01 : PMIOPort  Port=5  Side=Left  ConnectionType=Bus: ElectricalPower
  Bus Element Out1 : Outport  PortName=IF-BPR-SAF-01
  Bus Element Out2 : Outport  Port=2  PortName=IF-BPR-COM-01
  Bus Element Out3 : Outport  Port=3  PortName=IF-BPR-BVV-01

== system StarshipSystemModel/Starship/Propellent system/Booster propellant System/Pressurization, purge & venting/Pneumatic actuation gas COPVs ==
  IF-BNG-BHV-01 : PMIOPort  Side=Right  ConnectionType=Bus: PneumaticActuationGas
  IF-BNG-BPV-01 : PMIOPort  Port=2  Side=Right  ConnectionType=Bus: PneumaticActuationGas
  IF-BNG-BVC-01 : PMIOPort  Port=3  Side=Right  ConnectionType=Bus: PneumaticActuationGas
  IF-BNG-BVV-01 : PMIOPort  Port=4  Side=Right  ConnectionType=Bus: PneumaticActuationGas
  IF-BPQ-BNG-01 : PMIOPort  Port=5  Side=Left  ConnectionType=Bus: GroundPressurantSupply

== system StarshipSystemModel/Starship/Propellent system/Booster propellant System/Pressurization, purge & venting/Spin-start & igniter gas COPVs ==
  IF-BSG-BIG-01 : PMIOPort  Side=Right  ConnectionType=Bus: SpinStartIgniterGas
  IF-BPQ-BSG-01 : PMIOPort  Port=2  Side=Left  ConnectionType=Bus: GroundPressurantSupply

== system StarshipSystemModel/Starship/Propellent system/Booster propellant System/Pressurization, purge & venting/Vent & relief valves ==
  Bus Element In1 : Inport  PortName=IF-BPR-BVV-01
  IF-BFT-BVV-01 : PMIOPort  Side=Left  ConnectionType=Bus: AutogenousPressurantGas
  IF-BOT-BVV-01 : PMIOPort  Port=2  Side=Left  ConnectionType=Bus: AutogenousPressurantGas
  IF-BNG-BVV-01 : PMIOPort  Port=3  Side=Left  ConnectionType=Bus: PneumaticActuationGas

== system StarshipSystemModel/Starship/Propellent system/Ship propellant System/Feed & distribution/Distribution manifold ==
  IF-SDM-STP-01 : PMIOPort  Side=Right  ConnectionType=Bus: LiquidPropellantFeed
  IF-SHV-SDM-01 : PMIOPort  Port=2  Side=Left  ConnectionType=Bus: LiquidPropellantFeed
  IF-SPV-SDM-01 : PMIOPort  Port=3  Side=Left  ConnectionType=Bus: LiquidPropellantFeed

== system StarshipSystemModel/Starship/Propellent system/Ship propellant System/Feed & distribution/Feed controller ==
  Bus Element In1 : Inport  PortName=IF-GNC-SFC-01
  IF-PWR-SFC-01 : PMIOPort  Side=Left  ConnectionType=Bus: ElectricalPower
  Bus Element Out1 : Outport  PortName=IF-SFC-SPV-01
  Bus Element Out2 : Outport  Port=2  PortName=IF-SFC-SHV-01

== system StarshipSystemModel/Starship/Propellent system/Ship propellant System/Feed & distribution/Header tank switchover valve ==
  Bus Element In1 : Inport  PortName=IF-SFC-SHV-01
  IF-SLT-SHV-01 : PMIOPort  Side=Left  ConnectionType=Bus: LiquidPropellantFeed
  IF-SCH-SHV-01 : PMIOPort  Port=2  Side=Left  ConnectionType=Bus: LiquidPropellantFeed
  IF-SHV-SDM-01 : PMIOPort  Port=3  Side=Right  ConnectionType=Bus: LiquidPropellantFeed
  IF-SNG-SHV-01 : PMIOPort  Port=4  Side=Left  ConnectionType=Bus: PneumaticActuationGas

== system StarshipSystemModel/Starship/Propellent system/Ship propellant System/Feed & distribution/Main tank outlet valve (prevalve) ==
  Bus Element In1 : Inport  PortName=IF-SFC-SPV-01
  IF-SNG-SPV-01 : PMIOPort  Side=Left  ConnectionType=Bus: PneumaticActuationGas
  IF-SOT-SPV-01 : PMIOPort  Port=2  Side=Left  ConnectionType=Bus: LiquidPropellantFeed
  IF-SFT-SPV-01 : PMIOPort  Port=3  Side=Left  ConnectionType=Bus: LiquidPropellantFeed
  IF-SPV-SDM-01 : PMIOPort  Port=4  Side=Right  ConnectionType=Bus: LiquidPropellantFeed

== system StarshipSystemModel/Starship/Propellent system/Ship propellant System/Ground propellant interface/CH4 quick-disconnect panel ==
  IF-GND-SCQ-01 : PMIOPort  Side=Left
  IF-SCQ-SFT-01 : PMIOPort  Port=2  Side=Right  ConnectionType=Bus: LiquidPropellantFeed

== system StarshipSystemModel/Starship/Propellent system/Ship propellant System/Ground propellant interface/LOX quick-disconnect panel ==
  IF-GND-SLQ-01 : PMIOPort  Side=Left
  IF-SLQ-SOT-01 : PMIOPort  Port=2  Side=Right  ConnectionType=Bus: LiquidPropellantFeed

== system StarshipSystemModel/Starship/Propellent system/Ship propellant System/Ground propellant interface/Purge//pressurant ground QD ==
  IF-GND-SPQ-01 : PMIOPort  Side=Left  ConnectionType=Bus: GroundPressurantSupply
  IF-SPQ-SSG-01 : PMIOPort  Port=2  Side=Right  ConnectionType=Bus: GroundPressurantSupply
  IF-SPQ-SPR-01 : PMIOPort  Port=3  Side=Right  ConnectionType=Bus: GroundPressurantSupply
  IF-SPQ-SNG-01 : PMIOPort  Port=4  Side=Right  ConnectionType=Bus: GroundPressurantSupply

== system StarshipSystemModel/Starship/Propellent system/Ship propellant System/Pressurization, purge & venting/Autogenous pressurization regulator ==
  Bus Element In1 : Inport  PortName=IF-GNC-SPR-01
  IF-SPR-RVM-01 : PMIOPort  Side=Right  ConnectionType=Bus: CombustionGasFeed
  IF-STP-SPR-01 : PMIOPort  Port=2  Side=Left  ConnectionType=Bus: AutogenousPressurantGas
  IF-SPR-SOT-01 : PMIOPort  Port=3  Side=Right  ConnectionType=Bus: AutogenousPressurantGas
  IF-SPR-SFT-01 : PMIOPort  Port=4  Side=Right  ConnectionType=Bus: AutogenousPressurantGas
  IF-SPQ-SPR-01 : PMIOPort  Port=5  Side=Left  ConnectionType=Bus: GroundPressurantSupply
  IF-PWR-SPR-01 : PMIOPort  Port=6  Side=Left  ConnectionType=Bus: ElectricalPower
  Bus Element Out1 : Outport  PortName=IF-SPR-SAF-01
  Bus Element Out2 : Outport  Port=2  PortName=IF-SPR-STA-01
  Bus Element Out3 : Outport  Port=3  PortName=IF-SPR-SVV-01

== system StarshipSystemModel/Starship/Propellent system/Ship propellant System/Pressurization, purge & venting/Pneumatic actuation gas COPVs ==
  IF-SNG-SPV-01 : PMIOPort  Side=Right  ConnectionType=Bus: PneumaticActuationGas
  IF-SNG-SHV-01 : PMIOPort  Port=2  Side=Right  ConnectionType=Bus: PneumaticActuationGas
  IF-SNG-SVC-01 : PMIOPort  Port=3  Side=Right  ConnectionType=Bus: PneumaticActuationGas
  IF-SNG-SVV-01 : PMIOPort  Port=4  Side=Right  ConnectionType=Bus: PneumaticActuationGas
  IF-SPQ-SNG-01 : PMIOPort  Port=5  Side=Left  ConnectionType=Bus: GroundPressurantSupply

== system StarshipSystemModel/Starship/Propellent system/Ship propellant System/Pressurization, purge & venting/Spin-start & igniter gas COPVs ==
  IF-SSG-SIG-01 : PMIOPort  Side=Right  ConnectionType=Bus: SpinStartIgniterGas
  IF-SPQ-SSG-01 : PMIOPort  Port=2  Side=Left  ConnectionType=Bus: GroundPressurantSupply

== system StarshipSystemModel/Starship/Propellent system/Ship propellant System/Pressurization, purge & venting/Vent & relief valves ==
  Bus Element In1 : Inport  PortName=IF-SPR-SVV-01
  IF-SOT-SVV-01 : PMIOPort  Side=Left
  IF-SFT-SVV-01 : PMIOPort  Port=2  Side=Left
  IF-SNG-SVV-01 : PMIOPort  Port=3  Side=Left  ConnectionType=Bus: PneumaticActuationGas

== system StarshipSystemModel/Starship/Propellent system/Ship propellant System/Ship propellant tanks/Anti-slosh baffles ==

== system StarshipSystemModel/Starship/Propellent system/Ship propellant System/Ship propellant tanks/CH4 header tank ==
  IF-SCH-SHV-01 : PMIOPort  Side=Right  ConnectionType=Bus: LiquidPropellantFeed

== system StarshipSystemModel/Starship/Propellent system/Ship propellant System/Ship propellant tanks/CH4 main tank ==
  IF-SFT-SPV-01 : PMIOPort  Side=Right  ConnectionType=Bus: LiquidPropellantFeed
  IF-SPR-SFT-01 : PMIOPort  Port=2  Side=Left  ConnectionType=Bus: AutogenousPressurantGas
  IF-SFT-SVV-01 : PMIOPort  Port=3  Side=Right
  IF-SCQ-SFT-01 : PMIOPort  Port=4  Side=Left  ConnectionType=Bus: LiquidPropellantFeed

== system StarshipSystemModel/Starship/Propellent system/Ship propellant System/Ship propellant tanks/CH4 transfer tube (downcomer) ==

== system StarshipSystemModel/Starship/Propellent system/Ship propellant System/Ship propellant tanks/Common dome ==

== system StarshipSystemModel/Starship/Propellent system/Ship propellant System/Ship propellant tanks/LOX header tank ==
  IF-SLT-SHV-01 : PMIOPort  Side=Right  ConnectionType=Bus: LiquidPropellantFeed

== system StarshipSystemModel/Starship/Propellent system/Ship propellant System/Ship propellant tanks/LOX main tank ==
  IF-SOT-SPV-01 : PMIOPort  Side=Right  ConnectionType=Bus: LiquidPropellantFeed
  IF-SOT-PRS-01 : PMIOPort  Port=2  Side=Left  ConnectionType=Bus: StructuralLoad
  IF-SPR-SOT-01 : PMIOPort  Port=3  Side=Left  ConnectionType=Bus: AutogenousPressurantGas
  IF-SOT-SVV-01 : PMIOPort  Port=4  Side=Right
  IF-SLQ-SOT-01 : PMIOPort  Port=5  Side=Left  ConnectionType=Bus: LiquidPropellantFeed
